simulink subsystem "FT_Sensor_6D"  (R2025b)
settings: Solver=VariableStepAuto  StartTime=0.0  StopTime=10.0  RelTol=1e-3
values from neighbouring files (symbols this model uses):
  alpha = 1 - exp(-2*pi*fc/Fs)    [setup_handguiding_lab.m]
  bias_est = zeros(6,1)    [setup_handguiding_lab.m]
  cfg = ft_lab_config()    [setup_handguiding_lab.m]
undefined symbols (not defined in the file or in its folder): aButter, bButter, dspblkCoreblockFVToolHelper, gcbh
libraries: simulink x1
settings Model: Creator=Compu  LastModifiedBy=Compu

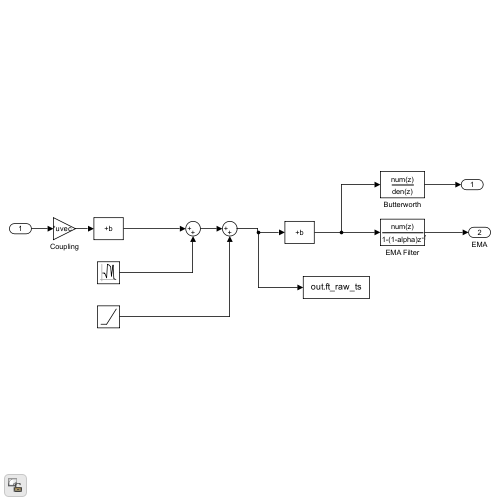
[thumbnail: Simulink's stored preview of the top-level diagram]
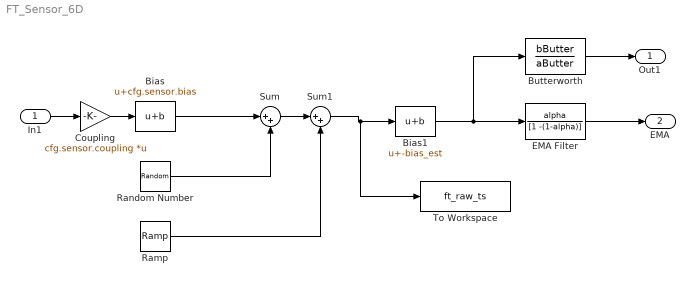
== system FT_Sensor_6D ==
  In1 : Inport
  Bias : Bias  Bias=cfg.sensor.bias  SaturateOnIntegerOverflow=off
  Bias1 : Bias  Bias=-bias_est  SaturateOnIntegerOverflow=off
  Butterworth : DiscreteFilter  LoadFcn=dspblkCoreblockFVToolHelper(gcbh,'load');  Numerator=bButter  Denominator=aButter
      settings: CopyFcn=dspblkCoreblockFVToolHelper(gcbh,'copy');  DeleteFcn=dspblkCoreblockFVToolHelper(gcbh,'close');  ModelCloseFcn=dspblkCoreblockFVToolHelper(gcbh,'close');  PreSaveFcn=dspblkCoreblockFVToolHelper(gcbh,'presave');  PostSaveFcn=dspblkCoreblockFVToolHelper(gcbh,'postsave');  CloseFcn=dspblkCoreblockFVToolHelper(gcbh,'close');
  Coupling : Gain  Gain=cfg.sensor.coupling  Multiplication=Matrix(K*u) (u vector)
  EMA Filter : DiscreteFilter  LoadFcn=dspblkCoreblockFVToolHelper(gcbh,'load');  Numerator=alpha  Denominator=[1 -(1-alpha)]
      settings: CopyFcn=dspblkCoreblockFVToolHelper(gcbh,'copy');  DeleteFcn=dspblkCoreblockFVToolHelper(gcbh,'close');  ModelCloseFcn=dspblkCoreblockFVToolHelper(gcbh,'close');  PreSaveFcn=dspblkCoreblockFVToolHelper(gcbh,'presave');  PostSaveFcn=dspblkCoreblockFVToolHelper(gcbh,'postsave');  CloseFcn=dspblkCoreblockFVToolHelper(gcbh,'close');
  Ramp : simulink/Sources/Ramp  slope=cfg.sensor.drift_per_s  start=0  InitialOutput=zeros(6,1)
  Random Number : RandomNumber  Mean=zeros(6,1)  Variance=cfg.sensor.noise_std.^2  Seed=[17;18;19;20;21;22]  SampleTime=0.002
  Sum : Sum  Inputs=|++
  Sum1 : Sum  Inputs=|++
  To Workspace : ToWorkspace  VariableName=ft_raw_ts  SaveFormat=Timeseries  SampleTime=-1
  Out1 : Outport
  EMA : Outport  Port=2
  wires:
  Bias1/1 -> EMA Filter/1, Butterworth/1
  Butterworth/1 -> Out1/1
  EMA Filter/1 -> EMA/1
  Bias/1 -> Sum/1
  Random Number/1 -> Sum/2
  Sum/1 -> Sum1/1
  Ramp/1 -> Sum1/2
  Sum1/1 -> Bias1/1, To Workspace/1
  In1/1 -> Coupling/1
  Coupling/1 -> Bias/1
